simulink model "My_gfm_battery_sil_12_ConvIGBT_zDomain"  (R2025b)
settings: Solver=ode23t  StartTime=0.0  StopTime=10  MaxStep=1e-4  RelTol=1e-3
PreLoadFcn:
  | close all;
  | clear all;
  | clc;
  | 
  | 
  | modelDir = fileparts(get_param(bdroot,'FileName'));
  | 
  | load_system(fullfile(modelDir,'controls_element_lib.slx'));
  | load_system(fullfile(modelDir,'test_sequence_lib.slx'));
  | 
  | Simulink.importExternalCTypes('.\circuitControls\circuitControls_A_autogen.h')
InitFcn:
  | % frequency nominals
  | F_NOM = 60;
  | W_NOM = 2 * pi * F_NOM;
  | 
  | % base values relative to inverter
  | % --------------------------------
  | VLL_INV_NOM = 480;
  | P_INV_NOM = 1e6;
  | Q_INV_NOM = 0.5e6;
  | S_INV_NOM = sqrt(P_INV_NOM^2 + Q_INV_NOM^2);
  | 
  | I_INV_BASE = S_INV_NOM/(sqrt(3)*VLL_INV_NOM);
  | Z_INV_BASE = VLL_INV_NOM^2/S_INV_NOM;
  | L_INV_BASE = Z_INV_BASE / W_NOM;
  | C_INV_BASE = 1 / (Z_INV_BASE * W_NOM);
  | 
  | % nominal ratings for power system model
  | % --------------------------------------
  | INVERTER_COUNT = 100;
  | 
  | VLV_NOM = VLL_INV_NOM;
  | VMV_NOM = 35e3;
  | VHV_NOM = 230e3;
  | S_PLANT = INVERTER_COUNT * S_INV_NOM;
  | 
  | N_GSU = VHV_NOM/VMV_NOM;
  | N_MVT = VMV_NOM/VLV_NOM;
  | 
  | I_LV_BASE = S_PLANT/(sqrt(3)*VLV_NOM);
  | I_MV_BASE = S_PLANT/(sqrt(3)*VMV_NOM);
  | I_HV_BASE = S_PLANT/(sqrt(3)*VHV_NOM);
  | 
  | Z_LV_BASE = VLV_NOM^2/S_PLANT;
  | Z_MV_BASE = VMV_NOM^2/S_PLANT;
  | Z_HV_BASE = VHV_NOM^2/S_PLANT;
  | 
  | L_LV_BASE = Z_LV_BASE / W_NOM;
  | L_MV_BASE = Z_MV_BASE / W_NOM;
  | L_HV_BASE = Z_HV_BASE / W_NOM;
  | C_LV_BASE = 1 / (Z_LV_BASE * W_NOM);
  | C_MV_BASE = 1 / (Z_MV_BASE * W_NOM);
  | C_HV_BASE = 1 / (Z_HV_BASE * W_NOM);
undefined symbols (not defined in the file): D1, D11, Delta, gcbh, j, SampleTime, sps_rtmsupport, Ts
libraries: simulink x56, spsVoltageMeasurementLib x21, spsThreePhaseSeriesRLCBranchLib x20, spsControlledCurrentSourceLib x20, spsControlledVoltageSourceLib x15, spsThreePhaseVIMeasurementLib x12, spsSeriesRLCBranchLib x11, spsGroundLib x11, test_sequence_lib x10, controls_element_lib x8, spsCurrentMeasurementLib x8, spsThreePhaseTransformerTwoWindingsLib x6
(part 1 of 9)
settings Model: SimulationMode=accelerator  Creator=HussamAlatrash  LastModifiedBy=ahhei
settings SolverCC: ZeroCrossControl=DisableAll  AlgebraicLoopSolver=TrustRegion
settings OptimizationCC: EfficientMapNaN2IntZero=off
settings DebuggingCC: ArithmeticOperatorsInVariantConditions=warning
settings HardwareCC: TargetBitPerPointer=64.0  TargetBitPerSizeT=64.0  TargetBitPerPtrDiffT=64.0  TargetLongLongMode=on  TargetIntDivRoundTo=Zero  TargetEndianess=LittleEndian  TargetWordSize=64.0  TargetHWDeviceType=MATLAB Host  ProdEqTarget=off
settings SFSimCC: CustomCodeUndefinedFunction=UseInterfaceOnly
settings RTWCC: GPUComputeCapability=3.5
settings CodeAppCC: MaxIdLength=128.0
settings GRTTargetCC: TargetLangStandard=C89/C90 (ANSI)  CombineOutputUpdateFcns=off  GRTInterface=on

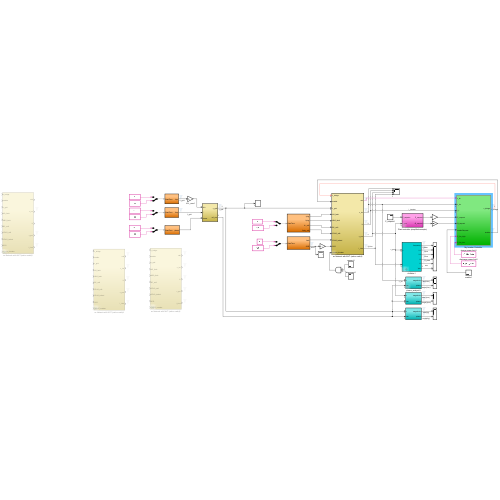
[thumbnail: Simulink's stored preview of the top-level diagram]
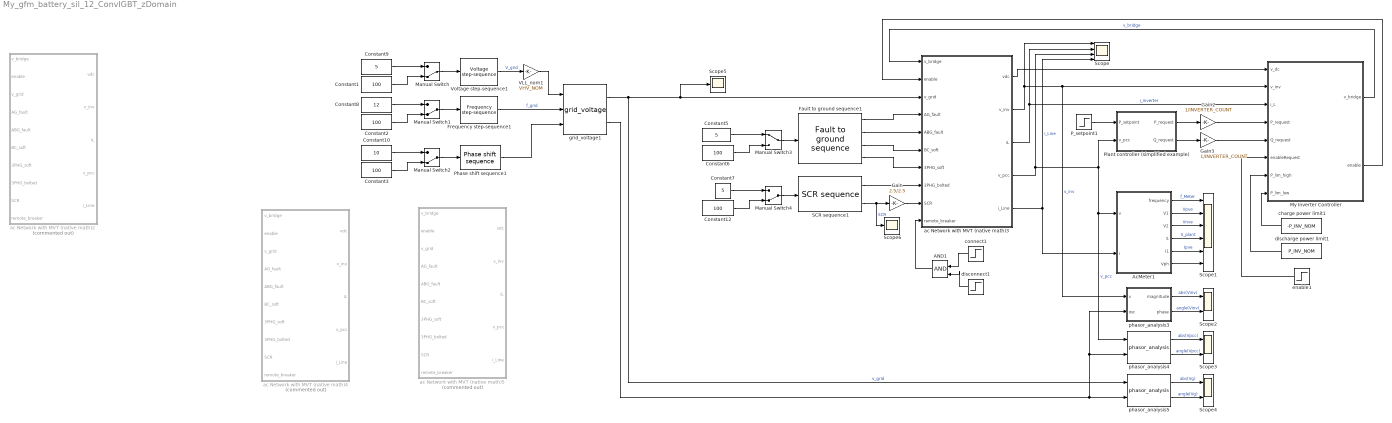
== system My_gfm_battery_sil_12_ConvIGBT_zDomain ==
  AND1 : Logic  IconShape=distinctive  AllPortsSameDT=off  OutDataTypeStr=boolean
  AcMeter1 : Subsystem  AncestorBlock=test_sequence_lib/AcMeter  mask{VllRated=VHV_NOM}
      mask prompts: VllRated "Rated line voltage"
  Constant{1..3,6,12} (5 alike) : Constant  Value=100
  Constant10 : Constant  Value=10
  Constant5 : Constant  Value=5
  Constant7 : Constant  Value=5
  Constant8 : Constant  Value=12
  Constant9 : Constant  Value=5
  Fault to ground sequence1 : test_sequence_lib/Fault to ground sequence  SystemSampleTime=-1  VariantActivationTime=update diagram  EmptyChoice=off  PassThrough=off  PassThroughVariantControl=(default)  EmptyChoiceVariantControl=(default)  AllowFlexibleInterface=on  Latency=0  AutoFrameSizeCalculation=off
  Frequency step-sequence1 : test_sequence_lib/Frequency step-sequence  SystemSampleTime=-1  VariantActivationTime=update diagram  EmptyChoice=off  PassThrough=off  PassThroughVariantControl=(default)  EmptyChoiceVariantControl=(default)  AllowFlexibleInterface=on  Latency=0  AutoFrameSizeCalculation=off
  Gain : Gain  Gain=2.5/2.5
  Gain2 : Gain  Gain=1/INVERTER_COUNT
  Gain3 : Gain  Gain=1/INVERTER_COUNT
  Manual Switch{,1..2,4} (4 alike) : ManualSwitch  CurrentSetting=0
  Manual Switch3 : ManualSwitch
  "My Inverter Controller " : Subsystem
  P_setpoint1 : Step  Time=4  After=S_PLANT*0.9  SampleTime=0
  Phase shift sequence1 : test_sequence_lib/Phase shift sequence  SystemSampleTime=-1  VariantActivationTime=update diagram  EmptyChoice=off  PassThrough=off  PassThroughVariantControl=(default)  EmptyChoiceVariantControl=(default)  AllowFlexibleInterface=on  Latency=0  AutoFrameSizeCalculation=off
  Plant controller (simplified example) : Subsystem  AncestorBlock=controls_element_lib/Battery plant controller
  SCR sequence1 : test_sequence_lib/SCR sequence  SystemSampleTime=-1  VariantActivationTime=update diagram  EmptyChoice=off  PassThrough=off  PassThroughVariantControl=(default)  EmptyChoiceVariantControl=(default)  AllowFlexibleInterface=on  Latency=0  AutoFrameSizeCalculation=off
  Scope : Scope  NumInputPorts=4
      settings: ActiveDisplayYMinimum=-650.914616267671  ActiveDisplayYMaximum=782.63422511063141
  Scope1 : Scope  NumInputPorts=6
      settings: ActiveDisplayYMinimum=59.77662  ActiveDisplayYMaximum=60.25431
  Scope2 : Scope  NumInputPorts=2
      settings: ActiveDisplayYMinimum=-67.80599  ActiveDisplayYMaximum=578.83849
  Scope3 : Scope  NumInputPorts=2
      settings: ActiveDisplayYMinimum=-24126.74884  ActiveDisplayYMaximum=239397.43913  DataLoggingVariableName=ScopeData2
  Scope4 : Scope  NumInputPorts=2
      settings: ActiveDisplayYMinimum=-28750  ActiveDisplayYMaximum=258750  DataLoggingVariableName=ScopeData3
  Scope5 : Scope
      settings: ActiveDisplayYMinimum=-219898.87455  ActiveDisplayYMaximum=239491.77196  DataLoggingVariableName=ScopeData5
  Scope6 : Scope
      settings: ActiveDisplayYMinimum=0.3125  ActiveDisplayYMaximum=22.1875
  VLL_nom1 : Gain  Gain=VHV_NOM
  Voltage step-sequence1 : test_sequence_lib/Voltage step-sequence  SystemSampleTime=-1  VariantActivationTime=update diagram  EmptyChoice=off  PassThrough=off  PassThroughVariantControl=(default)  EmptyChoiceVariantControl=(default)  AllowFlexibleInterface=on  Latency=0  AutoFrameSizeCalculation=off
  ac Network with MVT (native math)2 : Subsystem  Commented=on  AncestorBlock=test_sequence_lib/ac Network with MVT (native math)
  ac Network with MVT (native math)3 : Subsystem  AncestorBlock=test_sequence_lib/ac Network with MVT (native math)
  ac Network with MVT (native math)4 : Subsystem  Commented=on  AncestorBlock=test_sequence_lib/ac Network with MVT (native math)
  ac Network with MVT (native math)5 : Subsystem  Commented=on  AncestorBlock=test_sequence_lib/ac Network with MVT (native math)
  charge power limit1 : Constant  Value=-P_INV_NOM
  connect1 : Step  Time=0  SampleTime=0
  discharge power limit1 : Constant  Value=P_INV_NOM
  disconnect1 : Step  Time=100  Before=1  After=0  SampleTime=0
  enable1 : Step  Time=0.5  SampleTime=0
  grid_voltage1 : test_sequence_lib/grid_voltage  SystemSampleTime=-1  VariantActivationTime=update diagram  EmptyChoice=off  PassThrough=off  PassThroughVariantControl=(default)  EmptyChoiceVariantControl=(default)  AllowFlexibleInterface=on  Latency=0  AutoFrameSizeCalculation=off
  phasor_analysis3 : Subsystem  AncestorBlock=test_sequence_lib/phasor_analysis
  phasor_analysis4 : test_sequence_lib/phasor_analysis  SystemSampleTime=-1  VariantActivationTime=update diagram  EmptyChoice=off  PassThrough=off  PassThroughVariantControl=(default)  EmptyChoiceVariantControl=(default)  AllowFlexibleInterface=on  Latency=0  AutoFrameSizeCalculation=off
  phasor_analysis5 : test_sequence_lib/phasor_analysis  SystemSampleTime=-1  VariantActivationTime=update diagram  EmptyChoice=off  PassThrough=off  PassThroughVariantControl=(default)  EmptyChoiceVariantControl=(default)  AllowFlexibleInterface=on  Latency=0  AutoFrameSizeCalculation=off
  wires:
  Voltage step-sequence1/1 -> VLL_nom1/1  "V_grid"
  Manual Switch/1 -> Voltage step-sequence1/1
  Fault to ground sequence1/2 -> ac Network with MVT (native math)3/5(ABG_fault)
  AND1/1 -> ac Network with MVT (native math)3/10(remote_breaker)
  AcMeter1/3(V2) -> Scope1/3  "Vnve"
  discharge power limit1/1 -> "My Inverter Controller "/7(P_lim_high)
  Fault to ground sequence1/3 -> ac Network with MVT (native math)3/6(BC_soft)
  AcMeter1/6(Vph) -> Scope1/6
  "My Inverter Controller "/1(v_bridge) -> ac Network with MVT (native math)3/1(v_bridge)  "v_bridge"
  AcMeter1/2(V1) -> Scope1/2  "Vpve"
  Plant controller (simplified example)/1(P_request) -> Gain2/1
  ac Network with MVT (native math)3/2(v_inv) -> phasor_analysis3/1(v), "My Inverter Controller "/2(v_inv), Scope/1  "v_inv"
  P_setpoint1/1 -> Plant controller (simplified example)/1(P_setpoint)
  phasor_analysis5/1 -> Scope4/1  "abs(Vg)"
  AcMeter1/5(I1) -> Scope1/5  "Ipve"
  Plant controller (simplified example)/2(Q_request) -> Gain3/1
  grid_voltage1/1 -> phasor_analysis5/1, ac Network with MVT (native math)3/3(v_grid), Scope5/1  "v_grid"
  SCR sequence1/1 -> ac Network with MVT (native math)3/8(3PHG_bolted)
  phasor_analysis3/1(magnitude) -> Scope2/1  "abs(Vinv)"
  AcMeter1/4(S) -> Scope1/4  "S_plant"
  ac Network with MVT (native math)3/5(i_Line) -> Scope/4, AcMeter1/2(i)  "i_Line"
  AcMeter1/1(frequency) -> Scope1/1  "f_Meter"
  VLL_nom1/1 -> grid_voltage1/1
  phasor_analysis3/2(phase) -> Scope2/2  "angle(Vinv)"
  SCR sequence1/2 -> Scope6/1, Gain/1  "SCR"
  ac Network with MVT (native math)3/3(iL) -> "My Inverter Controller "/3(i_L), Scope/2  "i_inverter"
  disconnect1/1 -> AND1/2
  Fault to ground sequence1/4 -> ac Network with MVT (native math)3/7(3PHG_soft)
  ac Network with MVT (native math)3/4(v_pcc) -> Scope/3, Plant controller (simplified example)/2(v_pcc), phasor_analysis4/1, AcMeter1/1(v)  "v_pcc"
  charge power limit1/1 -> "My Inverter Controller "/8(P_lim_low)
  enable1/1 -> "My Inverter Controller "/6(enableRequest)
  Frequency step-sequence1/1 -> grid_voltage1/2  "f_grid"
  Fault to ground sequence1/1 -> ac Network with MVT (native math)3/4(AG_fault)
  grid_voltage1/2 -> phasor_analysis4/2, phasor_analysis3/2(osc), phasor_analysis5/2
  phasor_analysis5/2 -> Scope4/2  "angle(Vg)"
  connect1/1 -> AND1/1
  Constant9/1 -> Manual Switch/1
  Constant1/1 -> Manual Switch/2
  Constant2/1 -> Manual Switch1/2
  Manual Switch1/1 -> Frequency step-sequence1/1
  Constant8/1 -> Manual Switch1/1
  Manual Switch2/1 -> Phase shift sequence1/1
  Constant3/1 -> Manual Switch2/2
  Constant10/1 -> Manual Switch2/1
  Constant6/1 -> Manual Switch3/2
  Constant5/1 -> Manual Switch3/1
  Manual Switch3/1 -> Fault to ground sequence1/1
  Constant7/1 -> Manual Switch4/1
  Constant12/1 -> Manual Switch4/2
  Manual Switch4/1 -> SCR sequence1/1
  phasor_analysis4/1 -> Scope3/1  "abs(Vpcc)"
  phasor_analysis4/2 -> Scope3/2  "angle(Vpcc)"
  Phase shift sequence1/1 -> grid_voltage1/3
  Gain2/1 -> "My Inverter Controller "/4(P_request)
  Gain/1 -> ac Network with MVT (native math)3/9(SCR)
  ac Network with MVT (native math)3/1(vdc) -> "My Inverter Controller "/1(v_dc)
  "My Inverter Controller "/2(enable) -> ac Network with MVT (native math)3/2(enable)
  Gain3/1 -> "My Inverter Controller "/5(Q_request)

== system My_gfm_battery_sil_12_ConvIGBT_zDomain/AcMeter1 ==
  v : Inport
  i : Inport  Port=2
  Conj : Math  Operator=conj  SignedPower=on
  PLL_3ph : Subsystem
  Product : Product
  RMS calculator : Subsystem
  Scope : Scope  NumInputPorts=3
      settings: ActiveDisplayYMinimum=-39244.38194  ActiveDisplayYMaximum=169816.53056  DataLoggingVariableName=ScopeData4
  Scope1 : Scope  NumInputPorts=4
      settings: ActiveDisplayYMinimum=-89308.87867  ActiveDisplayYMaximum=439040.97064  DataLoggingVariableName=ScopeData7
  Sum of Elements : Sum  Commented=through  Inputs=+
  overVnom : Gain  Gain=1/VllRated
  phasor_analysis : Subsystem
  phasor_analysis1 : Subsystem  AncestorBlock=test_sequence_lib/AcMeter/phasor_analysis
  sqrt(3) : Gain  Gain=sqrt(3)
  sqrt(3)1 : Gain  Gain=sqrt(3)
  frequency : Outport
  V1 : Outport  Port=2
  V2 : Outport  Port=3
  S : Outport  Port=4
  I1 : Outport  Port=5
  Vph : Outport  Port=6
  wires:
  RMS calculator/1(out[3]) -> Vph/1
  PLL_3ph/2(osc[3]) -> phasor_analysis/2(osc), phasor_analysis1/2(osc)
  phasor_analysis/1(perPh) -> Scope/1
  Sum of Elements/1 -> Scope1/4, S/1  "S"
  v/1 -> RMS calculator/1(in[3]), phasor_analysis/1(in), overVnom/1
  PLL_3ph/1(freq) -> frequency/1
  overVnom/1 -> PLL_3ph/1(ref)
  Conj/1 -> Scope1/2, Product/2
  Product/1 -> Scope1/3, Sum of Elements/1
  phasor_analysis/2(pve) -> Scope/2, Scope1/1, Product/1, sqrt(3)/1  "Vpve_LN"
  phasor_analysis/3(nve) -> Scope/3, sqrt(3)1/1
  phasor_analysis1/2(pve) -> I1/1, Conj/1  "Ipve"
  sqrt(3)1/1 -> V2/1  "Vnve_LL"
  i/1 -> phasor_analysis1/1(in)
  sqrt(3)/1 -> V1/1  "Vpve_LL"

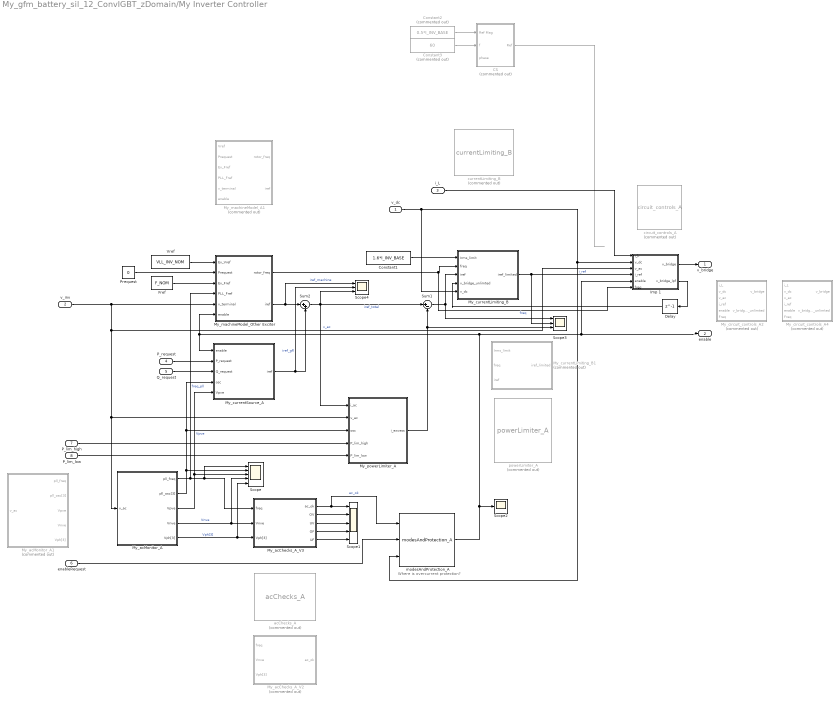
== system My_gfm_battery_sil_12_ConvIGBT_zDomain/My Inverter Controller  ==
  note: Where is overcurrent protection?
  v_dc : Inport
  v_inv : Inport  Port=2
  i_L : Inport  Port=3
  P_request : Inport  Port=4
  Q_request : Inport  Port=5
  enableRequest : Inport  Port=6
  P_lim_high : Inport  Port=7
  P_lim_low : Inport  Port=8
  CS : Subsystem  Commented=on  AncestorBlock=test_sequence_lib/grid_voltage
  Constant1 : Constant  Value=1.6*I_INV_BASE
  Constant2 : Constant  Commented=on  Value=0.5*I_INV_BASE
  Constant3 : Constant  Commented=on  Value=60
  Delay : Delay  DelayLength=1  InitialCondition=0
  Fref : Constant  Value=F_NOM
  Imp 1 : Subsystem  TreatAsAtomicUnit=on  SystemSampleTime=50e-6
  My_acChecks_A_V2 : Subsystem  Commented=on  AncestorBlock=controls_element_lib/acChecks_A  mask{VllRated=VLL_INV_NOM, NominalFrequency=F_NOM, Ts=1e-3, Time1=2, Time2=0, VHi=1.15, VLo=0.85, FHi=62, FLo=58, VNeg=0.2, Time3=0, OV3=1.3, OV3_Time=0.02, OV3_en=1, OV2=1.25, OV2_Time=2, OV2_en=1, OV1=1.2, OV1_Time=20, OV1_en=1, UV1=0.81, UV1_Time=15, UV1_en=1, UV2=0.5, UV2_Time=5, UV2_en=1, UV3=0.2, UV3_Time=1, UV3_en=1, OF3=70, OF3_Time=0.2, OF3_en=1, OF2=65, OF2_Time=10, OF2_en=1, OF1=63, OF1_Time=30, OF1_en=1, UF1=56, UF1_Time=30, UF1_en=1, UF2=55, UF2_Time=10, UF2_en=1, UF3=50, UF3_Time=0.2, UF3_en=1}
      mask prompts: VllRated "Rated Line-to-Line Voltage (V)"; NominalFrequency "Nominal Line Frequency (Hz)"; Ts "Operating Sample Time (sec)"; Time1 "Connection Time (sec)"; Time2 "Connection Out-of-Condition Delay (sec)"; VHi "High Voltage Threshold (pu)"; VLo "Low Voltage Threshold (pu)"; FHi "High Frequency Threshold (Hz)"; FLo "Low Frequency Threshold (Hz)"; VNeg "Negative Sequence Voltage Threshold (pu)"; Time3 "Trip Out-of-Condition Delay (sec)"; OV3 "OV PickUp 3 (pu)"; OV3_Time "OV Time 3 (sec)"; OV3_en "OV Enable 3"; OV2 "OV PickUp 2 (pu)"; OV2_Time "OV Time 2 (sec)"; OV2_en "OV Enable 2"; OV1 "OV PickUp 1 (pu)"; OV1_Time "OV Time 1 (sec)"; OV1_en "OV Enable 1"; UV1 "UV PickUp 1 (pu)"; UV1_Time "UV Time 1 (sec)"; UV1_en "UV Enable 1"; UV2 "UV PickUp 2 (pu)"; UV2_Time "UV Time 2 (sec)"; UV2_en "UV Enable 2"; UV3 "UV PickUp 3 (pu)"; UV3_Time "UV Time 3 (sec)"; UV3_en "UV Enable 3"; OF3 "OF PickUp 3 (Hz)"; OF3_Time "OF Time 3 (pu)"; OF3_en "OF Enable 3"; OF2 "OF PickUp 2 (Hz)"; OF2_Time "OF Time 2 (pu)"; OF2_en "OF Enable 2"; OF1 "OF PickUp 1 (Hz)"; OF1_Time "OF Time 1 (pu)"; OF1_en "OF Enable 1"; UF1 "UF PickUp 1 (Hz)"; UF1_Time "UF Time 1 (sec)"; UF1_en "UF Enable 1"; UF2 "UF PickUp 2 (Hz)"; UF2_Time "UF Time 2 (sec)"; UF2_en "UF Enable 2"; UF3 "UF PickUp 3 (Hz)"; UF3_Time "UF Time 3 (sec)"; UF3_en "UF Enable 3"
      mask DialogControl DescGroupVar Prompt: ACChecks
      mask DialogControl DecsTextVar Prompt: Grid Checks for Connection and Tripping
      mask DialogControl ParameterGroupVar Prompt: General Parameters
      mask DialogControl Container11 Prompt: Connection Settings
      mask DialogControl Container20 Prompt: Thresholds
      mask DialogControl Container3 Prompt: Trip Settings
      mask DialogControl Container12 Prompt: General Parameters
      mask DialogControl Container15 Prompt: Over Voltage Settings
      mask DialogControl Container4 Prompt: Over Voltage
      mask DialogControl Container19 Prompt: Under Voltage Settings
      mask DialogControl Container7 Prompt: Under Voltage
      mask DialogControl Container17 Prompt: Over Frequency Settings
      mask DialogControl Container9 Prompt: Over Frequency
      mask DialogControl Container16 Prompt: Under Frequency Settings
      mask DialogControl Container10 Prompt: Under Frequency
  My_acChecks_A_V3 : Subsystem  AncestorBlock=controls_element_lib/acChecks_A  mask{VllRated=VLL_INV_NOM, NominalFrequency=F_NOM, Ts=1e-3, Time1=2, Time2=0, VHi=1.15, VLo=0.85, FHi=62, FLo=58, VNeg=0.2, Time3=0, OV3=1.3, OV3_Time=0.02, OV3_en=1, OV2=1.25, OV2_Time=2, OV2_en=1, OV1=1.2, OV1_Time=20, OV1_en=1, UV1=0.81, UV1_Time=15, UV1_en=1, UV2=0.5, UV2_Time=5, UV2_en=1, UV3=0.2, UV3_Time=1, UV3_en=1, OF3=70, OF3_Time=0.2, OF3_en=1, OF2=65, OF2_Time=10, OF2_en=1, OF1=63, OF1_Time=30, OF1_en=1, UF1=56, UF1_Time=30, UF1_en=1, UF2=55, UF2_Time=10, UF2_en=1, UF3=50, UF3_Time=0.2, UF3_en=1}
      mask prompts: VllRated "Rated Line-to-Line Voltage (V)"; NominalFrequency "Nominal Line Frequency (Hz)"; Ts "Operating Sample Time (sec)"; Time1 "Connection Time (sec)"; Time2 "Connection Out-of-Condition Delay (sec)"; VHi "High Voltage Threshold (pu)"; VLo "Low Voltage Threshold (pu)"; FHi "High Frequency Threshold (Hz)"; FLo "Low Frequency Threshold (Hz)"; VNeg "Negative Sequence Voltage Threshold (pu)"; Time3 "Trip Out-of-Condition Delay (sec)"; OV3 "OV PickUp 3 (pu)"; OV3_Time "OV Time 3 (sec)"; OV3_en "OV Enable 3"; OV2 "OV PickUp 2 (pu)"; OV2_Time "OV Time 2 (sec)"; OV2_en "OV Enable 2"; OV1 "OV PickUp 1 (pu)"; OV1_Time "OV Time 1 (sec)"; OV1_en "OV Enable 1"; UV1 "UV PickUp 1 (pu)"; UV1_Time "UV Time 1 (sec)"; UV1_en "UV Enable 1"; UV2 "UV PickUp 2 (pu)"; UV2_Time "UV Time 2 (sec)"; UV2_en "UV Enable 2"; UV3 "UV PickUp 3 (pu)"; UV3_Time "UV Time 3 (sec)"; UV3_en "UV Enable 3"; OF3 "OF PickUp 3 (Hz)"; OF3_Time "OF Time 3 (pu)"; OF3_en "OF Enable 3"; OF2 "OF PickUp 2 (Hz)"; OF2_Time "OF Time 2 (pu)"; OF2_en "OF Enable 2"; OF1 "OF PickUp 1 (Hz)"; OF1_Time "OF Time 1 (pu)"; OF1_en "OF Enable 1"; UF1 "UF PickUp 1 (Hz)"; UF1_Time "UF Time 1 (sec)"; UF1_en "UF Enable 1"; UF2 "UF PickUp 2 (Hz)"; UF2_Time "UF Time 2 (sec)"; UF2_en "UF Enable 2"; UF3 "UF PickUp 3 (Hz)"; UF3_Time "UF Time 3 (sec)"; UF3_en "UF Enable 3"
      mask DialogControl DescGroupVar Prompt: ACChecks
      mask DialogControl DecsTextVar Prompt: Grid Checks for Connection and Tripping
      mask DialogControl ParameterGroupVar Prompt: General Parameters
      mask DialogControl Container11 Prompt: Connection Settings
      mask DialogControl Container20 Prompt: Thresholds
      mask DialogControl Container3 Prompt: Trip Settings
      mask DialogControl Container12 Prompt: General Parameters
      mask DialogControl Container15 Prompt: Over Voltage Settings
      mask DialogControl Container4 Prompt: Over Voltage
      mask DialogControl Container19 Prompt: Under Voltage Settings
      mask DialogControl Container7 Prompt: Under Voltage
      mask DialogControl Container17 Prompt: Over Frequency Settings
      mask DialogControl Container9 Prompt: Over Frequency
      mask DialogControl Container16 Prompt: Under Frequency Settings
      mask DialogControl Container10 Prompt: Under Frequency
  My_acMonitor_A : Subsystem  AncestorBlock=controls_element_lib/acMonitor_A  InitFcn=Ts = 1000e-6;  TreatAsAtomicUnit=on  SystemSampleTime=1000e-6  mask{VllRated=VLL_INV_NOM, nominalFrequency=F_NOM}
      mask prompts: VllRated "Rated line-to-line voltage (V)"; nominalFrequency "Nominal line frequency (Hz)"
  My_acMonitor_A1 : Subsystem  Commented=on  AncestorBlock=controls_element_lib/acMonitor_A  mask{VllRated=VLL_INV_NOM, nominalFrequency=F_NOM}
      mask prompts: VllRated "Rated line-to-line voltage (V)"; nominalFrequency "Nominal line frequency (Hz)"
  My_circuit_controls_A2 : Subsystem  Commented=on  AncestorBlock=controls_element_lib/circuit_controls_A  InitFcn=Ts =200e-6;  TreatAsAtomicUnit=on  SystemSampleTime=200e-6
  My_circuit_controls_A4 : Subsystem  Commented=on  AncestorBlock=controls_element_lib/circuit_controls_A  InitFcn=Ts =200e-6;  TreatAsAtomicUnit=on  SystemSampleTime=200e-6
  My_currentLimiting_B : Subsystem  AncestorBlock=controls_element_lib/currentLimiting_B  TreatAsAtomicUnit=on  SystemSampleTime=Ts  mask{IRated=I_INV_BASE, peakSoftLimit=2.6, peakHardLimit=3.6, Ts=200e-6}
      mask prompts: IRated "Rated current (A)"; peakSoftLimit "Soft peak limit (pu)"; peakHardLimit "Hard peak limit (pu)"; Ts "Sample Time"
  My_currentLimiting_B1 : Subsystem  Commented=on  AncestorBlock=controls_element_lib/currentLimiting_B  mask{IRated=I_INV_BASE, peakSoftLimit=2.6, peakHardLimit=3.6}
      mask prompts: IRated "Rated current (A)"; peakSoftLimit "Soft peak limit (pu)"; peakHardLimit "Hard peak limit (pu)"
  My_currentSource_A : Subsystem  AncestorBlock=controls_element_lib/currentSource_A  InitFcn=Ts = 200e-6;  TreatAsAtomicUnit=on  SystemSampleTime=200e-6  mask{VllRated=VLL_INV_NOM, SRated=S_INV_NOM, nominalFrequency=F_NOM, Plimit=P_INV_NOM/S_INV_NOM, Qlimit=Q_INV_NOM/S_INV_NOM, CSOnline=1}
      mask prompts: VllRated "Rated line-to-line voltage (V)"; SRated "Rated power (VA)"; nominalFrequency "Nominal line frequency (Hz)"; Plimit "Real power request limit (pu)"; Qlimit "Reactive power request limit (pu)"; CSOnline "Current Source Online"
  My_machineModel_A1 : Subsystem  Commented=on  AncestorBlock=controls_element_lib/machineModel_A  mask{SRated=S_INV_NOM, VllRated=VLL_INV_NOM, nominalFrequency=F_NOM, inertialConstant=2.5, kDroop=1, kDamper=2, Xs=0.3, rs=0.08, Qlimit1=0.5, wExciter=10, FreqRefSel=1, MachOnline=0}
      mask prompts: SRated "Rated power (VA)"; VllRated "Rated Voltage (Volts, line-to-line)"; nominalFrequency "Nominal frequency (Hz)"; inertialConstant "Inertial constant (seconds)"; kDroop "Droop gain (pu/Hz)"; kDamper "Damper gain (pu/Hz)"; Xs "Stator reactance (pu)"; rs "Stator resistance (pu)"; Qlimit1 "Reactive power request limit (pu)"; wExciter "Exciter Bandwidth (rad)"; FreqRefSel "Frequency Reference Selector"; MachOnline "Machine Online"
      mask DialogControl DescGroupVar Prompt: Machine Model and Controls
  My_machineModel_Other Exciter : Subsystem  AncestorBlock=controls_element_lib/machineModel_A  TreatAsAtomicUnit=on  SystemSampleTime=Ts  mask{SRated=S_INV_NOM, VllRated=VLL_INV_NOM, nominalFrequency=F_NOM, MachOnline=1, inertialConstant=2.5, kDamper=2, tau_damp=0.3, Xs=0.3, rs=0.08, rn=0, wExciter=10, VoltRefSel=0, Kpv=10, tpv=0.05, kpq=0.1, kiq=1, Qleak=10e-3, FreqRefSel=1, kDroop=1, wGoverner=1/0.3, kpSync=20, kpFastSync=1, wSync=2*pi*50, kpSyncFade=4, SyncFadeThres=0.2, tauMeas=0.02, tauBkSt=0.5, Ts=200e-6}
      mask prompts: SRated "Rated power (VA)"; VllRated "Rated Voltage (Volts, line-to-line)"; nominalFrequency "Nominal frequency (Hz)"; MachOnline "Machine Online"; inertialConstant "Inertial constant (seconds)"; kDamper "Damper gain (pu/Hz)"; tau_damp "Damper time constant (sec)"; Xs "Stator reactance (pu)"; rs "Stator resistance (pu)"; rn "Neutral resistance (pu)"; wExciter "Exciter Bandwidth (rad)"; VoltRefSel "Voltage Reference Selector"; Kpv "Voltage proportional gain (pu Q/ pu v)"; tpv "Voltage proportional LPF time constant (sec)"; kpq "Reactive power proportional gain"; kiq "Reactive power Integral gain"; Qleak "Leakage"; FreqRefSel "Frequency Reference Selector"; kDroop "Droop gain (pu/Hz)"; wGoverner "Governer Bandwidth (rad/s)"; kpSync "Synchronizer proportional gain (pu P / pu V)"; kpFastSync "Fast synchronizer gain (pu P / pu V)"; wSync "Synchronizer HPF Bandwidth(rad/s)"; kpSyncFade "Synchronizer fade gain (pu P/ puV)"; SyncFadeThres "Synchronizer fade threshold (pu)"; tauMeas "Measurements filters time constant (sec)"; tauBkSt "Black Start filter time constant (sec)"; Ts "Sample Time"
      mask DialogControl DescGroupVar Prompt: Machine Model and Controls
      mask DialogControl ParameterGroupVar Prompt: Ratings
      mask DialogControl Container3 Prompt: Machine Parameters
      mask DialogControl Container4 Prompt: Mechanical Parameters
      mask DialogControl Container5 Prompt: Electrical Parameters
      mask DialogControl Container7 Prompt: AVR Parameters
      mask DialogControl Container6 Prompt: Governer Parameters
      mask DialogControl Container9 Prompt: Synchronizer Parameters
  My_powerLimiter_A : Subsystem  AncestorBlock=controls_element_lib/powerLimiter_A  TreatAsAtomicUnit=on  SystemSampleTime=Ts  mask{VllRated=VLL_INV_NOM, nominalFrequency=F_NOM, wPowerLimiter=3, Ts=200e-6}
      mask prompts: VllRated "Rated line-to-line voltage (V)"; nominalFrequency "Nominal line frequency (Hz)"; wPowerLimiter "Bandwidth (rad)"; Ts "Sample Time"
  Prequest : Constant  Value=0
  Scope : Scope  NumInputPorts=5
      settings: ActiveDisplayYMinimum=58.2372  ActiveDisplayYMaximum=61.12702  DataLoggingVariableName=ScopeData8
  Scope1 : Scope  NumInputPorts=5
      settings: ActiveDisplayYMinimum=-0.125  ActiveDisplayYMaximum=1.125
  Scope2 : Scope
      settings: ActiveDisplayYMinimum=-0.125  ActiveDisplayYMaximum=1.125  DataLoggingVariableName=ScopeData2
  Scope3 : Scope  NumInputPorts=3
      settings: ActiveDisplayYMinimum=-2673.42252  ActiveDisplayYMaximum=2648.08579  DataLoggingVariableName=ScopeData3
  Scope4 : Scope  NumInputPorts=3
      settings: ActiveDisplayYMinimum=-1971.04314  ActiveDisplayYMaximum=2260.89044  DataLoggingVariableName=ScopeData4
  Sum1 : Sum  Inputs=|+-
  Sum2 : Sum  Inputs=|++
  Vref : Constant  Value=VLL_INV_NOM
  acChecks_A : controls_element_lib/acChecks_A  Commented=on  VllRated=VLL_INV_NOM  nominalFrequency=F_NOM  tRequalify=2  T_CNTL=1e-3
  circuit_controls_A : controls_element_lib/circuit_controls_A  Commented=on  SystemSampleTime=-1  VariantActivationTime=update diagram  EmptyChoice=off  PassThrough=off  PassThroughVariantControl=(default)  EmptyChoiceVariantControl=(default)  AllowFlexibleInterface=on  Latency=0  AutoFrameSizeCalculation=off
  currentLimiting_B : controls_element_lib/currentLimiting_B  Commented=on  IRated=I_INV_BASE  peakSoftLimit=2.6  peakHardLimit=3.6
  modesAndProtection_A : controls_element_lib/modesAndProtection_A  dcOvervotlageThreshold=1800  dcUndervotlageThreshold=700  dcTripClearTimeout=0.2
  powerLimiter_A : controls_element_lib/powerLimiter_A  Commented=on  VllRated=VLL_INV_NOM  nominalFrequency=F_NOM  wPowerLimiter=3
  v_bridge : Outport
  enable : Outport  Port=2
  wires:
  Vref/1 -> My_machineModel_Other Exciter/1(Ex_Vref)
  Prequest/1 -> My_machineModel_Other Exciter/2(Prequest)
  My_machineModel_Other Exciter/2(iref) -> Scope4/1, Sum2/1  "iref_machine"
  My_acMonitor_A/2(pll_osc[3]) -> Scope/2, My_currentSource_A/4(osc), My_powerLimiter_A/3(osc)
  My_currentLimiting_B/1(iref_limited) -> Imp 1/4(i_ref), Scope3/2  "i_ref"
  My_currentSource_A/1(iref) -> Sum2/2, Scope4/2  "iref_gfl"
  Sum2/1 -> Sum1/1, Scope4/3, My_powerLimiter_A/1(i_ac)  "iref_total"
  My_acMonitor_A/3(Vpve) -> My_currentSource_A/5(Vpve), Scope/3  "Vpve"
  Q_request/1 -> My_currentSource_A/3(Q_request)
  P_request/1 -> My_currentSource_A/2(P_request)
  enableRequest/1 -> modesAndProtection_A/2
  modesAndProtection_A/1 -> Scope2/1, My_machineModel_Other Exciter/6(enable), My_currentSource_A/1(enable), Imp 1/5(enable), enable/1
  My_acMonitor_A/5(Vph[3]) -> My_acChecks_A_V3/3(Vph[3]), Scope/5  "Vph[3]"
  My_acChecks_A_V3/1(ac_ok) -> Scope1/1, modesAndProtection_A/1  "ac_ok"
  Constant1/1 -> My_currentLimiting_B/1(Irms_limit)
  My_acMonitor_A/1(pll_freq) -> My_machineModel_Other Exciter/4(PLL_Fref), My_acChecks_A_V3/1(freq), Scope/1  "freq_pll"
  My_acMonitor_A/4(Vnve) -> My_acChecks_A_V3/2(Vnve), Scope/4  "Vnve"
  P_lim_low/1 -> My_powerLimiter_A/5(P_lim_low)
  P_lim_high/1 -> My_powerLimiter_A/4(P_lim_high)
  My_powerLimiter_A/1(i_excess) -> Sum1/2, Scope3/3
  Sum1/1 -> My_currentLimiting_B/3(iref), Scope3/1
  v_dc/1 -> Imp 1/2(v_dc), modesAndProtection_A/3, My_currentLimiting_B/5(v_dc)
  My_machineModel_Other Exciter/1(rotor_freq) -> Imp 1/6(freq), My_currentLimiting_B/2(freq)  "freq"
  v_inv/1 -> My_machineModel_Other Exciter/5(v_terminal), Imp 1/3(v_ac), My_acMonitor_A/1(v_ac), My_powerLimiter_A/2(v_ac)  "v_ac"
  Fref/1 -> My_machineModel_Other Exciter/3(Ex_Fref)
  My_acChecks_A_V3/2(OV) -> Scope1/2
  My_acChecks_A_V3/3(UV) -> Scope1/3
  My_acChecks_A_V3/4(OF) -> Scope1/4
  My_acChecks_A_V3/5(UF) -> Scope1/5
  Constant2/1 -> CS/1(Ref Mag)
  Constant3/1 -> CS/2(f)
  CS/1(Ref) -> ?
  Imp 1/1(v_bridge) -> v_bridge/1
  i_L/1 -> Imp 1/1(i_L)
  Imp 1/2(v_bridge_lpf) -> Delay/1
  Delay/1 -> My_currentLimiting_B/4(v_bridge_unlimted)

== system My_gfm_battery_sil_12_ConvIGBT_zDomain/Plant controller (simplified example) ==
  P_setpoint : Inport
  v_pcc : Inport  Port=2
  Gain : Gain  Gain=-1
  Gain1 : Gain  Gain=S_PLANT
  Gain2 : Gain  Gain=S_PLANT
  Gain4 : Gain  Gain=1/VHV_NOM
  LVRT_foldback : Subsystem
  Meter : Subsystem
  Saturation : Saturate  UpperLimit=0.9*S_PLANT  LowerLimit=-0.9*S_PLANT
  Saturation Dynamic : simulink/Discontinuities/Saturation Dynamic  OutMin=[]  OutMax=[]  OutDataTypeStr=Inherit: Same as second input  OutDataType=fixdt(1, 16)  OutScaling=2^-10  DoSatur=off
  Scope : Scope  NumInputPorts=5
      settings: ActiveDisplayYMinimum=-8.42781966139E+6  ActiveDisplayYMaximum=1.0713546508948E+8
  VoltVAr : Subsystem
  P_request : Outport
  Q_request : Outport  Port=2
  wires:
  Gain/1 -> Saturation Dynamic/3
  Saturation Dynamic/1 -> Scope/1, P_request/1  "P_request"
  LVRT_foldback/1(limit_pu) -> Scope/2, Gain2/1  "spinout_limit_Vpcc"
  Gain2/1 -> Saturation Dynamic/1, Gain/1
  Saturation/1 -> Saturation Dynamic/2
  Gain4/1 -> Scope/5, Meter/1(v)
  P_setpoint/1 -> Saturation/1
  v_pcc/1 -> Gain4/1
  Gain1/1 -> Q_request/1  "Q_request"
  Meter/1(Vpve) -> Scope/4, VoltVAr/1(Vpve_pu), LVRT_foldback/1(Vpve_pu)  "V_pu_plant"
  VoltVAr/1(Q) -> Gain1/1, Scope/3

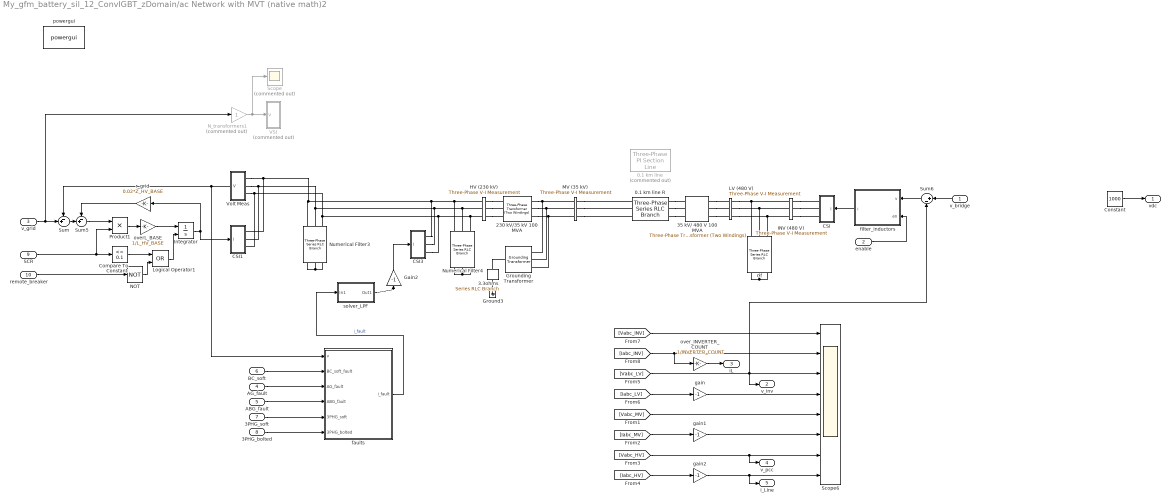
== system My_gfm_battery_sil_12_ConvIGBT_zDomain/ac Network with MVT (native math)2 ==
  v_bridge : Inport
  enable : Inport  Port=2
  v_grid : Inport  Port=3
  AG_fault : Inport  Port=4
  ABG_fault : Inport  Port=5
  BC_soft : Inport  Port=6
  3PHG_soft : Inport  Port=7
  3PHG_bolted : Inport  Port=8
  SCR : Inport  Port=9
  remote_breaker : Inport  Port=10
  0.1 km line : spsThreePhasePISectionLineLib/Three-Phase PI Section Line  Commented=on  LConnTagsString=a|b|c  RConnTagsString=A|B|C  Length=0.1  Frequency=60  Resistances=[0.1153 0.413]  Inductances=[1.05e-3 3.32e-3]  Capacitances=[11.33e-009 5.01e-009]
  0.1 km line R : spsThreePhaseSeriesRLCBranchLib/Three-Phase Series RLC Branch  LConnTagsString=A|B|C  RConnTagsString=A|B|C  BranchType=R  Resistance=0.001  Inductance=50e-6  Capacitance=0.03*C_LV_BASE  Measurements=None
  230 kV/35 kV 100 MVA : spsThreePhaseTransformerTwoWindingsLib/Three-Phase Transformer (Two Windings)  Winding1Connection=Yg  Winding2Connection=Delta (D1)  CoreType=Three single-phase transformers  SetSaturation=off  Hysteresis=off  DataFile='basic_model'  SetInitialFlux=off  Measurements=None  UNITS=pu  NominalPower=[S_PLANT F_NOM ]  Winding1="[ VHV_NOM  0.05/50   0.05 ]"  Winding2="[ VMV_NOM  0.05/50  0.05]"  Rm=500  Lm=500  L0=0.5  Saturation="[ 0,0  ;  0.005,1.2  ;  1.0,1.4 ]"  InitialFluxes=[ 0.8 , -0.8 , 0.7 ]  BreakLoop=off  DiscreteSolver=Trapezoidal iterative  DataType=off  TransfoNumber=0
  "3.3ohms " : spsSeriesRLCBranchLib/Series RLC Branch  LConnTagsString=__new0  RConnTagsString=__new0  BranchType=R  Resistance=3.3  Inductance=[]  SetiL0=off  InitialCurrent=0  Capacitance=[]  Setx0=off  InitialVoltage=0  Measurements=None
  35 kV/ 480 V 100 MVA : spsThreePhaseTransformerTwoWindingsLib/Three-Phase Transformer (Two Windings)  Winding1Connection=Delta (D11)  Winding2Connection=Yg  CoreType=Three single-phase transformers  SetSaturation=off  Hysteresis=off  DataFile='hysteresis'  SetInitialFlux=off  Measurements=None  UNITS=pu  NominalPower="[S_PLANT  F_NOM]"  Winding1=[VMV_NOM , 0.03/50 , 0.03]  Winding2=[ VLV_NOM, 0.03/50 , 0.03]  Rm=500  Lm=500  L0=0.5  Saturation=[ 0,0 ; 0.0024,1.2 ; 1.0,1.52 ]  InitialFluxes=[ 0.8 , -0.8 , 0.7 ]  BreakLoop=off  DiscreteSolver=Trapezoidal iterative  DataType=off  TransfoNumber=0
  CSI : Subsystem
  CSI1 : Subsystem
  CSI3 : Subsystem
  Cf : spsThreePhaseSeriesRLCBranchLib/Three-Phase Series RLC Branch  LConnTagsString=A|B|C  RConnTagsString=A|B|C  BranchType=C  Resistance=10  Inductance=1e-3  Capacitance=0.03*C_LV_BASE  Measurements=None
  Compare To Constant : simulink/Logic and Bit Operations/Compare To Constant  relop=<=  const=0.1  OutDataTypeStr=boolean
  Constant : Constant  Value=1000
  Gain2 : Gain  Gain=-1
  Ground3 : spsGroundLib/Ground  LConnTagsString=a
  "Grounding Transformer " : spsGroundingTransformerLib/Grounding Transformer   UNITS=pu  NominalPower="[S_PLANT  F_NOM]"  NominalVoltage=VMV_NOM  ZeroSequenceImpedance_pu=[0.025 0.75]  MagnetizationBranch_pu=[500 500]  ZeroSequenceImpedance_SI=[0.052083 589.05]  MagnetizationBranch_SI=[1041.7 3.927e+005]  Measurements=None
  HV (230 kV) : spsThreePhaseVIMeasurementLib/Three-Phase V-I Measurement  VoltageMeasurement=phase-to-ground  SetLabelV=on  LabelV=Vabc_HV  Vpu=off  VpuLL=off  CurrentMeasurement=yes  SetLabelI=on  LabelI=Iabc_HV  Ipu=off  Pbase=S_PLANT  Vbase=VHV_NOM  OutputType=Complex  PhasorSimulation=off  PSBequivalent=0
  INV (480 V) : spsThreePhaseVIMeasurementLib/Three-Phase V-I Measurement  VoltageMeasurement=phase-to-ground  SetLabelV=on  LabelV=Vabc_INV  Vpu=off  VpuLL=off  CurrentMeasurement=yes  SetLabelI=on  LabelI=Iabc_INV  Ipu=off  Pbase=S_INV_NOM  Vbase=VLV_NOM  OutputType=Complex  PhasorSimulation=off  PSBequivalent=0
  Integrator : Integrator  ExternalReset=level
  LV (480 V) : spsThreePhaseVIMeasurementLib/Three-Phase V-I Measurement  VoltageMeasurement=phase-to-ground  SetLabelV=on  LabelV=Vabc_LV  Vpu=off  VpuLL=off  CurrentMeasurement=yes  SetLabelI=on  LabelI=Iabc_LV  Ipu=off  Pbase=S_INV_NOM  Vbase=VLV_NOM  OutputType=Complex  PhasorSimulation=off  PSBequivalent=0
  Logical Operator1 : Logic  Operator=OR  AllPortsSameDT=off  OutDataTypeStr=boolean
  MV (35 kV) : spsThreePhaseVIMeasurementLib/Three-Phase V-I Measurement  VoltageMeasurement=phase-to-ground  SetLabelV=on  LabelV=Vabc_MV  Vpu=off  VpuLL=off  CurrentMeasurement=yes  SetLabelI=on  LabelI=Iabc_MV  Ipu=off  Pbase=S_INV_NOM  Vbase=VMV_NOM  OutputType=Complex  PhasorSimulation=off  PSBequivalent=0
  NOT : Logic  Operator=NOT  IconShape=distinctive  AllPortsSameDT=off  OutDataTypeStr=boolean
  N_transformers1 : Gain  Commented=on
  Numerical Filter3 : spsThreePhaseSeriesRLCBranchLib/Three-Phase Series RLC Branch  LConnTagsString=A|B|C  RConnTagsString=A|B|C  BranchType=R  Resistance=50*Z_HV_BASE  Inductance=50e-6  Capacitance=0.03*C_LV_BASE  Measurements=None
  Numerical Filter4 : spsThreePhaseSeriesRLCBranchLib/Three-Phase Series RLC Branch  LConnTagsString=A|B|C  RConnTagsString=A|B|C  BranchType=R  Resistance=50*Z_HV_BASE  Inductance=50e-6  Capacitance=0.03*C_LV_BASE  Measurements=None
  Product1 : Product
  Scope : Scope  Commented=on
      settings: ActiveDisplayYMinimum=-35721.72542  ActiveDisplayYMaximum=35721.72542
  Scope6 : Scope  NumInputPorts=8
      settings: ActiveDisplayYMinimum=-1  ActiveDisplayYMaximum=1  DataLoggingVariableName=ScopeData6
  Sum : Sum  Inputs=-+|
  Sum5 : Sum  Inputs=-+|
  Sum6 : Sum  Inputs=|+-
  VSI : Subsystem  Commented=on
  Volt Meas : Subsystem
  faults : Subsystem
  filter_inductors : Subsystem
  gain : Gain  Gain=-1
  gain1 : Gain  Gain=-1
  gain2 : Gain  Gain=-1
  overL_BASE : Gain  Gain=1/L_HV_BASE
  over_INVERTER_COUNT : Gain  Gain=-1/INVERTER_COUNT
  powergui : spspowerguiLib/powergui  Priority=2  SimulationMode=Continuous  SampleTime=0  frequency=60  Iterations=50  frequencyindice=0  Pbase=100e6  ErrMax=1e-4  UnitsV=kV  UnitsW=MW  buscounter=0  FunctionMessages=off  echomessages=off  EnableUseOfTLC=off  CurrentSourceSwitches=off  DisableSnubberDevices=on  DisableRonSwitches=off  DisableVfSwitches=off  DisplayEquations=off  AutomaticDiscreteSolvers=off  SolverType=Tustin  Interpol=off  ExternalGateDelay=off  methode=off  Ts=0  x0status=blocks  SPID=on  SwTol=0  HookPort=off  NonlinearTolerance=1e-4  nMaxIteration=100  ContinueOnMaxIteration=off  RestoreLinks=warning  ResistiveCurrentMeasurement=off  Frange=[0:2:500]  Ylog=off  Xlog=on  ShowGrid=off  save=off  variable=ZData  structure=0  ZoomFFT=on  StartTime=0.0  cycles=1  DisplayStyle=1  fundamental=60  FreqAxis=off  MaxFrequency=1000  frequencyindicesteady=1  RmsSteady=1  display=off
  r_grid : Gain  Gain=0.02*Z_HV_BASE
  solver_LPF : Subsystem
  vdc : Outport
  v_inv : Outport  Port=2
  iL : Outport  Port=3
  v_pcc : Outport  Port=4
  i_Line : Outport  Port=5
  wires:
  AG_fault/1 -> faults/3(AG_fault)
  ABG_fault/1 -> faults/4(ABG_fault)
  BC_soft/1 -> faults/2(BC_soft_fault)
  overL_BASE/1 -> Integrator/1
  Integrator/1 -> CSI1/1(I), r_grid/1
  faults/1(i_fault) -> solver_LPF/1(In1)  "i_fault"
  3PHG_bolted/1 -> faults/6(3PHG_bolted)
  Product1/1 -> overL_BASE/1
  r_grid/1 -> Sum5/1
  Sum5/1 -> Product1/1
  Sum/1 -> Sum5/2
  3PHG_soft/1 -> faults/5(3PHG_soft)
  Volt Meas/1(V) -> faults/1(v), Sum/1
  solver_LPF/1(Out1) -> Gain2/1
  [Vabc_LV] -> Sum6/2, v_inv/1, Scope6/3
  [Vabc_HV] -> v_pcc/1, Scope6/7
  [Vabc_INV] -> Scope6/1
  [Iabc_LV] -> gain/1
  [Vabc_MV] -> Scope6/5
  v_bridge/1 -> Sum6/1
  Sum6/1 -> filter_inductors/1(v)
  enable/1 -> filter_inductors/2(en)
  Constant/1 -> vdc/1
  filter_inductors/1(i) -> CSI/1(I)
  [Iabc_INV] -> over_INVERTER_COUNT/1, Scope6/2
  v_grid/1 -> N_transformers1/1, Sum/2
  N_transformers1/1 -> Scope/1, VSI/1(V)
  over_INVERTER_COUNT/1 -> iL/1
  gain/1 -> Scope6/4
  [Iabc_HV] -> gain2/1
  [Iabc_MV] -> gain1/1
  gain1/1 -> Scope6/6
  gain2/1 -> i_Line/1, Scope6/8
  Gain2/1 -> CSI3/1(I)
  NOT/1 -> Logical Operator1/2
  Compare To Constant/1 -> Logical Operator1/1
  Logical Operator1/1 -> Integrator/2
  remote_breaker/1 -> NOT/1
  SCR/1 -> Compare To Constant/1, Product1/2
  connections:
  "Grounding Transformer "/LConn1 -- 230 kV/35 kV 100 MVA/RConn1 -- MV (35 kV)/LConn1
  "Grounding Transformer "/LConn2 -- 230 kV/35 kV 100 MVA/RConn2 -- MV (35 kV)/LConn2
  "Grounding Transformer "/LConn3 -- 230 kV/35 kV 100 MVA/RConn3 -- MV (35 kV)/LConn3
  "3.3ohms "/LConn1 -- "Grounding Transformer "/RConn1
  MV (35 kV)/RConn3 -- 0.1 km line R/LConn3
  MV (35 kV)/RConn2 -- 0.1 km line R/LConn2
  "3.3ohms "/RConn1 -- Ground3/LConn1
  MV (35 kV)/RConn1 -- 0.1 km line R/LConn1
  Cf/RConn2 -- Cf/RConn1 -- Cf/RConn3
  LV (480 V)/RConn1 -- Cf/LConn1 -- INV (480 V)/LConn1
  LV (480 V)/RConn2 -- Cf/LConn2 -- INV (480 V)/LConn2
  HV (230 kV)/RConn1 -- 230 kV/35 kV 100 MVA/LConn1
  HV (230 kV)/RConn2 -- 230 kV/35 kV 100 MVA/LConn2
  HV (230 kV)/RConn3 -- 230 kV/35 kV 100 MVA/LConn3
  LV (480 V)/RConn3 -- Cf/LConn3 -- INV (480 V)/LConn3
  35 kV/ 480 V 100 MVA/RConn1 -- LV (480 V)/LConn1
  35 kV/ 480 V 100 MVA/RConn2 -- LV (480 V)/LConn2
  35 kV/ 480 V 100 MVA/RConn3 -- LV (480 V)/LConn3
  INV (480 V)/RConn1 -- CSI/RConn1
  INV (480 V)/RConn2 -- CSI/RConn2
  INV (480 V)/RConn3 -- CSI/RConn3
  0.1 km line R/RConn2 -- 35 kV/ 480 V 100 MVA/LConn2
  0.1 km line R/RConn1 -- 35 kV/ 480 V 100 MVA/LConn1
  0.1 km line R/RConn3 -- 35 kV/ 480 V 100 MVA/LConn3
  Numerical Filter3/RConn2 -- Numerical Filter3/RConn1 -- Numerical Filter3/RConn3
  Numerical Filter4/RConn2 -- Numerical Filter4/RConn1 -- Numerical Filter4/RConn3
  Volt Meas/LConn2 -- Numerical Filter3/LConn2 -- Numerical Filter4/LConn2 -- HV (230 kV)/LConn2 -- CSI3/RConn2 -- CSI1/RConn2
  Numerical Filter4/LConn1 -- HV (230 kV)/LConn1 -- CSI3/RConn1 -- Numerical Filter3/LConn1 -- Volt Meas/LConn1 -- CSI1/RConn1
  Numerical Filter4/LConn3 -- HV (230 kV)/LConn3 -- CSI3/RConn3 -- Numerical Filter3/LConn3 -- Volt Meas/LConn3 -- CSI1/RConn3

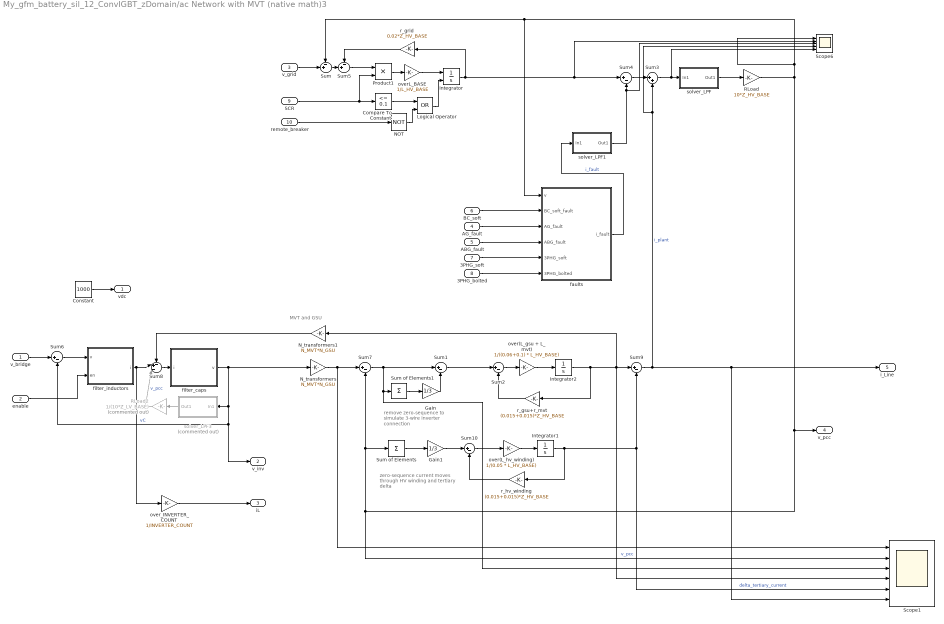
== system My_gfm_battery_sil_12_ConvIGBT_zDomain/ac Network with MVT (native math)3 ==
  note: zero-sequence current moves through HV winding and tertiary delta
  note: remove zero-sequence to simulate 3-wire inverter connection
  note: MVT and GSU
  v_bridge : Inport
  enable : Inport  Port=2
  v_grid : Inport  Port=3
  AG_fault : Inport  Port=4
  ABG_fault : Inport  Port=5
  BC_soft : Inport  Port=6
  3PHG_soft : Inport  Port=7
  3PHG_bolted : Inport  Port=8
  SCR : Inport  Port=9
  remote_breaker : Inport  Port=10
  Compare To Constant : simulink/Logic and Bit Operations/Compare To Constant  relop=<=  const=0.1  OutDataTypeStr=boolean
  Constant : Constant  Value=1000
  Gain : Gain  Gain=1/3
  Gain1 : Gain  Gain=1/3
  Integrator : Integrator  ExternalReset=level
  Integrator1 : Integrator
  Integrator2 : Integrator
  Logical Operator : Logic  Operator=OR  AllPortsSameDT=off  OutDataTypeStr=boolean
  NOT : Logic  Operator=NOT  IconShape=distinctive  AllPortsSameDT=off  OutDataTypeStr=boolean
  N_transformers : Gain  Gain=N_MVT*N_GSU
  N_transformers1 : Gain  Gain=N_MVT*N_GSU
  Product1 : Product
  RLoad : Gain  Gain=10*Z_HV_BASE
  RLoad2 : Gain  Commented=on  Gain=1/(10*Z_LV_BASE)
  Scope1 : Scope  NumInputPorts=6
      settings: ActiveDisplayYMinimum=-446429.70138  ActiveDisplayYMaximum=455812.19957  DataLoggingVariableName=ScopeData7
  Scope6 : Scope  NumInputPorts=5
      settings: ActiveDisplayYMinimum=-0.10239  ActiveDisplayYMaximum=0.12997  DataLoggingVariableName=ScopeData6
  Sum : Sum  Inputs=-+|
  Sum of Elements : Sum  Inputs=+
  Sum of Elements1 : Sum  Inputs=+
  Sum{1..2,4,6..7,9..10} (7 alike) : Sum  Inputs=|+-
  Sum3 : Sum  Inputs=|++
  Sum5 : Sum  Inputs=-+|
  Sum8 : Sum  Inputs=-+-|
  faults : Subsystem
  filter_caps : Subsystem
  filter_inductors : Subsystem
  over(L_gsu + L_mvt) : Gain  Gain=1/((0.06+0.1) * L_HV_BASE)
  over(L_hv_winding) : Gain  Gain=1/(0.05 * L_HV_BASE)
  overL_BASE : Gain  Gain=1/L_HV_BASE
  over_INVERTER_COUNT : Gain  Gain=1/INVERTER_COUNT
  r_grid : Gain  Gain=0.02*Z_HV_BASE
  r_gsu+r_mvt : Gain  Gain=(0.015+0.015)*Z_HV_BASE
  r_hv_winding : Gain  Gain=(0.015+0.015)*Z_HV_BASE
  solver_LPF : Subsystem
  solver_LPF1 : Subsystem
  solver_LPF3 : Subsystem  Commented=on
  vdc : Outport
  v_inv : Outport  Port=2
  iL : Outport  Port=3
  v_pcc : Outport  Port=4
  i_Line : Outport  Port=5
  wires:
  AG_fault/1 -> faults/3(AG_fault)
  ABG_fault/1 -> faults/4(ABG_fault)
  BC_soft/1 -> faults/2(BC_soft_fault)
  Gain1/1 -> Sum10/1
  Sum of Elements/1 -> Gain1/1
  Sum10/1 -> over(L_hv_winding)/1
  r_hv_winding/1 -> Sum10/2
  Integrator1/1 -> r_hv_winding/1, Scope1/5, Sum9/2  "delta_tertiary_current"
  over(L_hv_winding)/1 -> Integrator1/1
  Sum9/1 -> Scope1/6, i_Line/1, Scope6/4, Sum3/2  "i_plant"
  N_transformers1/1 -> Sum8/1
  N_transformers/1 -> Scope1/1, Sum7/1
  over_INVERTER_COUNT/1 -> iL/1
  filter_caps/1(v) -> N_transformers/1, solver_LPF3/1(In1), Sum6/2, v_inv/1  "vC"
  Sum8/1 -> filter_caps/1(i)
  filter_inductors/1(i) -> over_INVERTER_COUNT/1, Sum8/2
  enable/1 -> filter_inductors/2(en)
  Sum6/1 -> filter_inductors/1(v)
  r_gsu+r_mvt/1 -> Sum2/2
  Sum1/1 -> Sum2/1
  Gain/1 -> Sum1/2
  Sum of Elements1/1 -> Gain/1
  Sum2/1 -> over(L_gsu + L_mvt)/1
  Sum7/1 -> Sum1/1, Scope1/3, Sum of Elements1/1
  over(L_gsu + L_mvt)/1 -> Integrator2/1
  solver_LPF/1(Out1) -> RLoad/1
  remote_breaker/1 -> NOT/1
  overL_BASE/1 -> Integrator/1
  Integrator/1 -> Scope6/2, Sum4/1, r_grid/1
  solver_LPF1/1(Out1) -> Scope6/3, Sum4/2
  RLoad/1 -> Sum of Elements/1, Sum7/2, Scope1/2, v_pcc/1, Sum/1, faults/1(v), Scope6/1  "v_pcc"
  faults/1(i_fault) -> solver_LPF1/1(In1)  "i_fault"
  3PHG_bolted/1 -> faults/6(3PHG_bolted)
  v_bridge/1 -> Sum6/1
  Product1/1 -> overL_BASE/1
  SCR/1 -> Compare To Constant/1, Product1/2
  r_grid/1 -> Sum5/1
  Sum3/1 -> Scope6/5, solver_LPF/1(In1)
  Sum4/1 -> Sum3/1
  v_grid/1 -> Sum/2
  Sum5/1 -> Product1/1
  Sum/1 -> Sum5/2
  Integrator2/1 -> Scope1/4, Sum9/1, N_transformers1/1, r_gsu+r_mvt/1
  3PHG_soft/1 -> faults/5(3PHG_soft)
  solver_LPF3/1(Out1) -> RLoad2/1
  Constant/1 -> vdc/1
  Compare To Constant/1 -> Logical Operator/1
  NOT/1 -> Logical Operator/2
  Logical Operator/1 -> Integrator/2
  RLoad2/1 -> Sum8/3  "v_pcc"
